simulink model "boost_cascade_pi_average"  (R2025a)
settings: Solver=ode23tb  StartTime=0.0  StopTime=0.5  MaxStep=5e-06  RelTol=1e-05
PreLoadFcn:
  | if ~exist('BM', 'var'), boost_mrac_params; end
InitFcn:
  | if ~exist('BM', 'var'), boost_mrac_params; end
undefined symbols (not defined in the file): BM, DiscIntNeverNeededParam
Description:
  | DC-DC boost converter, cascade PI (Fig. 9, Eqs. 42-43), state-space averaged model (Eqs. 3-9). Recreation of Yanarates & Zhou, IEEE Access 10 (2022) 44909. Parameters: struct BM from boost_mrac_params.m.
settings Model: Creator=runner  LastModifiedBy=runner
settings DataIOCC: SaveOutput=off  SignalLogging=off  SaveTime=off
settings DebuggingCC: AlgebraicLoopMsg=error

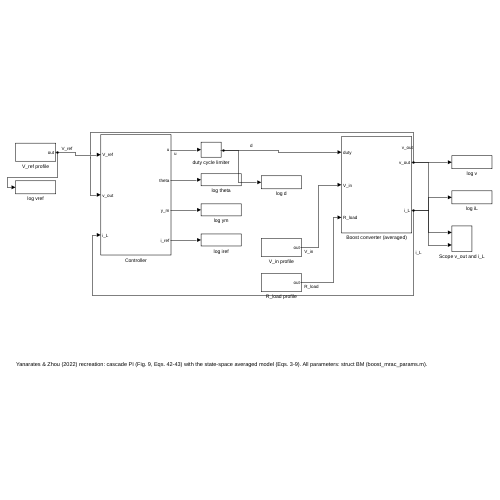
[thumbnail: Simulink's stored preview of the top-level diagram]
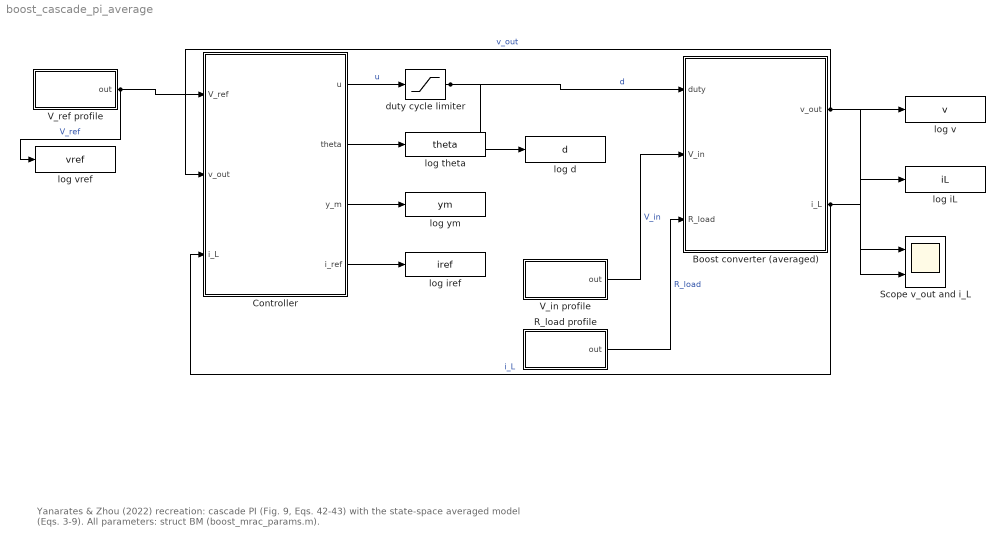
== system boost_cascade_pi_average ==
  note: Yanarates & Zhou (2022) recreation: cascade PI (Fig. 9, Eqs. 42-43) with the state-space averaged model (Eqs. 3-9). All parameters: struct BM (boost_mrac_params.m).
  Boost converter (averaged) : Subsystem
  Controller : Subsystem
  R_load profile : Subsystem
  Scope v_out and i_L : Scope  NumInputPorts=2
  V_in profile : Subsystem
  V_ref profile : Subsystem
  duty cycle limiter : Saturate  UpperLimit=BM.dmax  LowerLimit=BM.dmin
  log d : ToWorkspace  VariableName=d  SaveFormat=Timeseries  SampleTime=BM.Ts
  log iL : ToWorkspace  VariableName=iL  SaveFormat=Timeseries  SampleTime=BM.Ts
  log iref : ToWorkspace  VariableName=iref  SaveFormat=Timeseries  SampleTime=BM.Ts
  log theta : ToWorkspace  VariableName=theta  SaveFormat=Timeseries  SampleTime=BM.Ts
  log v : ToWorkspace  VariableName=v  SaveFormat=Timeseries  SampleTime=BM.Ts
  log vref : ToWorkspace  VariableName=vref  SaveFormat=Timeseries  SampleTime=BM.Ts
  log ym : ToWorkspace  VariableName=ym  SaveFormat=Timeseries  SampleTime=BM.Ts
  wires:
  V_ref profile/1(out) -> Controller/1(V_ref), log vref/1  "V_ref"
  Controller/1(u) -> duty cycle limiter/1  "u"
  duty cycle limiter/1 -> Boost converter (averaged)/1(duty), log d/1  "d"
  V_in profile/1(out) -> Boost converter (averaged)/2(V_in)  "V_in"
  R_load profile/1(out) -> Boost converter (averaged)/3(R_load)  "R_load"
  Boost converter (averaged)/1(v_out) -> Controller/2(v_out), log v/1, Scope v_out and i_L/1  "v_out"
  Boost converter (averaged)/2(i_L) -> Controller/3(i_L), log iL/1, Scope v_out and i_L/2  "i_L"
  Controller/2(theta) -> log theta/1
  Controller/3(y_m) -> log ym/1
  Controller/4(i_ref) -> log iref/1

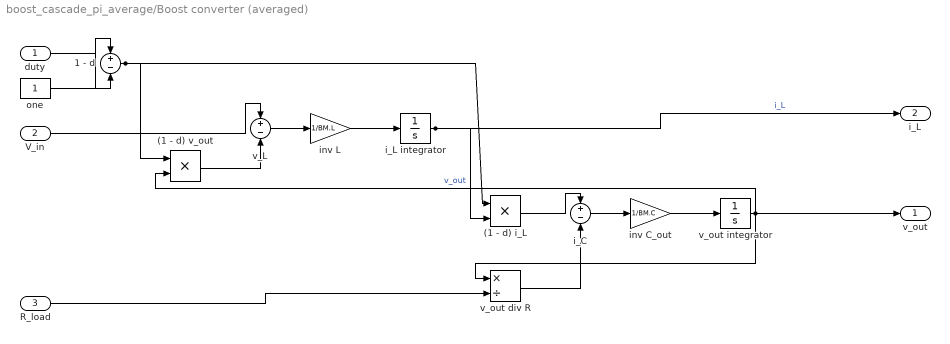
== system boost_cascade_pi_average/Boost converter (averaged) ==
  duty : Inport
  V_in : Inport  Port=2
  R_load : Inport  Port=3
  (1 - d) i_L : Product  Inputs=**
  (1 - d) v_out : Product  Inputs=**
  1 - d : Sum  Inputs=+-
  i_C : Sum  Inputs=+-
  i_L integrator : Integrator  InitialCondition=BM.iL0  LimitOutput=on  LowerSaturationLimit=BM.iL_min
  inv C_out : Gain  Gain=1/BM.C
  inv L : Gain  Gain=1/BM.L
  one : Constant
  v_L : Sum  Inputs=+-
  v_out div R : Product  Inputs=*/
  v_out integrator : Integrator  InitialCondition=BM.v0
  v_out : Outport
  i_L : Outport  Port=2
  wires:
  one/1 -> 1 - d/1
  duty/1 -> 1 - d/2
  1 - d/1 -> (1 - d) v_out/1, (1 - d) i_L/1
  v_out integrator/1 -> (1 - d) v_out/2, v_out div R/1, v_out/1  "v_out"
  V_in/1 -> v_L/1
  (1 - d) v_out/1 -> v_L/2
  v_L/1 -> inv L/1
  inv L/1 -> i_L integrator/1
  i_L integrator/1 -> (1 - d) i_L/2, i_L/1  "i_L"
  R_load/1 -> v_out div R/2
  (1 - d) i_L/1 -> i_C/1
  v_out div R/1 -> i_C/2
  i_C/1 -> inv C_out/1
  inv C_out/1 -> v_out integrator/1

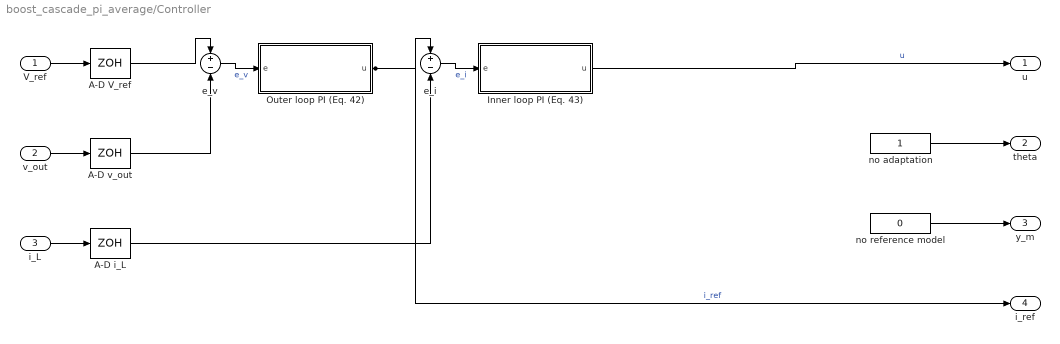
== system boost_cascade_pi_average/Controller ==
  V_ref : Inport
  v_out : Inport  Port=2
  i_L : Inport  Port=3
  A-D V_ref : ZeroOrderHold  SampleTime=BM.Ts
  A-D i_L : ZeroOrderHold  SampleTime=BM.Ts
  A-D v_out : ZeroOrderHold  SampleTime=BM.Ts
  Inner loop PI (Eq. 43) : Subsystem
  Outer loop PI (Eq. 42) : Subsystem
  e_i : Sum  Inputs=+-
  e_v : Sum  Inputs=+-
  no adaptation : Constant
  no reference model : Constant  Value=0
  u : Outport
  theta : Outport  Port=2
  y_m : Outport  Port=3
  i_ref : Outport  Port=4
  wires:
  V_ref/1 -> A-D V_ref/1
  v_out/1 -> A-D v_out/1
  i_L/1 -> A-D i_L/1
  A-D v_out/1 -> e_v/2
  e_v/1 -> Outer loop PI (Eq. 42)/1(e)  "e_v"
  Outer loop PI (Eq. 42)/1(u) -> e_i/1, i_ref/1  "i_ref"
  A-D i_L/1 -> e_i/2
  e_i/1 -> Inner loop PI (Eq. 43)/1(e)  "e_i"
  A-D V_ref/1 -> e_v/1
  Inner loop PI (Eq. 43)/1(u) -> u/1  "u"
  no adaptation/1 -> theta/1
  no reference model/1 -> y_m/1

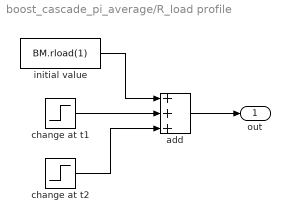
== system boost_cascade_pi_average/R_load profile ==
  add : Sum  Inputs=+++
  change at t1 : Step  Time=BM.t_rload(1)  After=BM.rload(2)-BM.rload(1)  SampleTime=0
  change at t2 : Step  Time=BM.t_rload(2)  After=BM.rload(3)-BM.rload(2)  SampleTime=0
  initial value : Constant  Value=BM.rload(1)
  out : Outport
  wires:
  initial value/1 -> add/1
  change at t1/1 -> add/2
  change at t2/1 -> add/3
  add/1 -> out/1

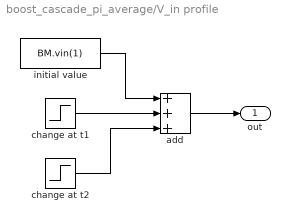
== system boost_cascade_pi_average/V_in profile ==
  add : Sum  Inputs=+++
  change at t1 : Step  Time=BM.t_vin(1)  After=BM.vin(2)-BM.vin(1)  SampleTime=0
  change at t2 : Step  Time=BM.t_vin(2)  After=BM.vin(3)-BM.vin(2)  SampleTime=0
  initial value : Constant  Value=BM.vin(1)
  out : Outport
  wires:
  initial value/1 -> add/1
  change at t1/1 -> add/2
  change at t2/1 -> add/3
  add/1 -> out/1

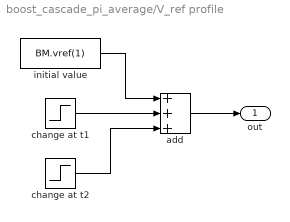
== system boost_cascade_pi_average/V_ref profile ==
  add : Sum  Inputs=+++
  change at t1 : Step  Time=BM.t_vref(1)  After=BM.vref(2)-BM.vref(1)  SampleTime=0
  change at t2 : Step  Time=BM.t_vref(2)  After=BM.vref(3)-BM.vref(2)  SampleTime=0
  initial value : Constant  Value=BM.vref(1)
  out : Outport
  wires:
  initial value/1 -> add/1
  change at t1/1 -> add/2
  change at t2/1 -> add/3
  add/1 -> out/1

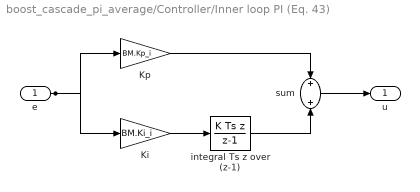
== system boost_cascade_pi_average/Controller/Inner loop PI (Eq. 43) ==
  e : Inport
  Ki : Gain  Gain=BM.Ki_i
  Kp : Gain  Gain=BM.Kp_i
  integral Ts z over (z-1) : DiscreteIntegrator  IntegratorMethod=Integration: Backward Euler  gainval=1  SampleTime=BM.Ts  ICPrevOutput=DiscIntNeverNeededParam  ICPrevScaledInput=DiscIntNeverNeededParam
  sum : Sum
  u : Outport
  wires:
  e/1 -> Kp/1, Ki/1
  Ki/1 -> integral Ts z over (z-1)/1
  Kp/1 -> sum/1
  integral Ts z over (z-1)/1 -> sum/2
  sum/1 -> u/1

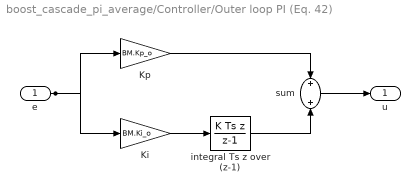
== system boost_cascade_pi_average/Controller/Outer loop PI (Eq. 42) ==
  e : Inport
  Ki : Gain  Gain=BM.Ki_o
  Kp : Gain  Gain=BM.Kp_o
  integral Ts z over (z-1) : DiscreteIntegrator  IntegratorMethod=Integration: Backward Euler  gainval=1  SampleTime=BM.Ts  ICPrevOutput=DiscIntNeverNeededParam  ICPrevScaledInput=DiscIntNeverNeededParam
  sum : Sum
  u : Outport
  wires:
  e/1 -> Kp/1, Ki/1
  Ki/1 -> integral Ts z over (z-1)/1
  Kp/1 -> sum/1
  integral Ts z over (z-1)/1 -> sum/2
  sum/1 -> u/1
